simulink model "Exp7"  (R2025b)
settings: Solver=VariableStepAuto  StartTime=0.0  StopTime=10.0  RelTol=1e-3
libraries: simulink x4
settings Model: Creator=SUBHASH  LastModifiedBy=SUBHASH

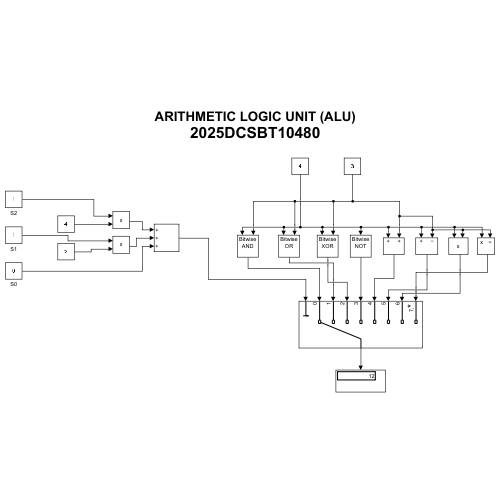
[thumbnail: Simulink's stored preview of the top-level diagram]
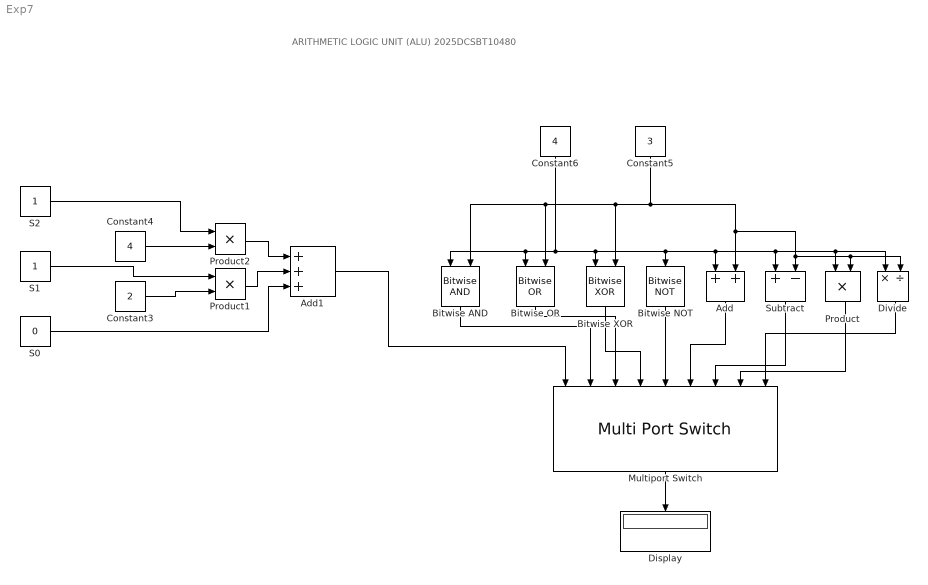
== system Exp7 ==
  note: ARITHMETIC LOGIC UNIT (ALU)
      | 2025DCSBT10480
  Add : Sum
  Add1 : Sum  Inputs=+++
  Bitwise AND : simulink/Logic and Bit Operations/Bitwise Operator  logicop=AND  UseBitMask=off  NumInputPorts=2  BitMask=bin2dec('11011001')  BitMaskRealWorld=Stored Integer
      settings: LibrarySourceBlock=|
      | simulink/Quick Insert/Logic and Bit
      | Operations/Bitwise AND
  Bitwise NOT : simulink/Logic and Bit Operations/Bitwise Operator  logicop=NOT  UseBitMask=off  BitMask=bin2dec('11011001')  BitMaskRealWorld=Stored Integer
      settings: LibrarySourceBlock=|
      | simulink/Quick Insert/Logic and Bit
      | Operations/Bitwise NOT
  Bitwise OR : simulink/Logic and Bit Operations/Bitwise Operator  logicop=OR  UseBitMask=off  NumInputPorts=2  BitMask=bin2dec('11011001')  BitMaskRealWorld=Stored Integer
      settings: LibrarySourceBlock=|
      | simulink/Quick Insert/Logic and Bit
      | Operations/Bitwise OR
  Bitwise XOR : simulink/Logic and Bit Operations/Bitwise Operator  logicop=XOR  UseBitMask=off  NumInputPorts=2  BitMask=bin2dec('11011001')  BitMaskRealWorld=Stored Integer
      settings: LibrarySourceBlock=|
      | simulink/Quick Insert/Logic and Bit
      | Operations/Bitwise XOR
  Constant3 : Constant  Value=2
  Constant4 : Constant  Value=4
  Constant5 : Constant  Value=3  OutDataTypeStr=uint8
  Constant6 : Constant  Value=4  OutDataTypeStr=uint8
  Display : Display
  Divide : Product  Inputs=*/
  Multiport Switch : MultiPortSwitch  DataPortOrder=Zero-based contiguous  Inputs=8  zeroidx=on  SaturateOnIntegerOverflow=off  InputSameDT=off
  Product : Product
  Product1 : Product
  Product2 : Product
  S0 : Constant  Value=0
  S1 : Constant
  S2 : Constant
  Subtract : Sum  Inputs=+-
  wires:
  S1/1 -> Product1/1
  Constant3/1 -> Product1/2
  S2/1 -> Product2/1
  Constant4/1 -> Product2/2
  S0/1 -> Add1/3
  Product1/1 -> Add1/2
  Product2/1 -> Add1/1
  Add1/1 -> Multiport Switch/1
  Constant6/1 -> Subtract/1, Product/1, Divide/1, Add/1, Bitwise NOT/1, Bitwise XOR/1, Bitwise AND/1, Bitwise OR/1
  Constant5/1 -> Add/2, Product/2, Divide/2, Subtract/2, Bitwise XOR/2, Bitwise AND/2, Bitwise OR/2
  Bitwise AND/1 -> Multiport Switch/2
  Bitwise OR/1 -> Multiport Switch/3
  Bitwise XOR/1 -> Multiport Switch/4
  Bitwise NOT/1 -> Multiport Switch/5
  Add/1 -> Multiport Switch/6
  Subtract/1 -> Multiport Switch/7
  Product/1 -> Multiport Switch/8
  Divide/1 -> Multiport Switch/9
  Multiport Switch/1 -> Display/1
